simulink model "Q3 – Ramp Signal Folding"  (R2024b)
settings: Solver=FixedStepAuto  StartTime=-5  StopTime=5  FixedStep=0.001  RelTol=1e-3
libraries: simulink x1
settings Model: Creator=sobha  LastModifiedBy=sobha

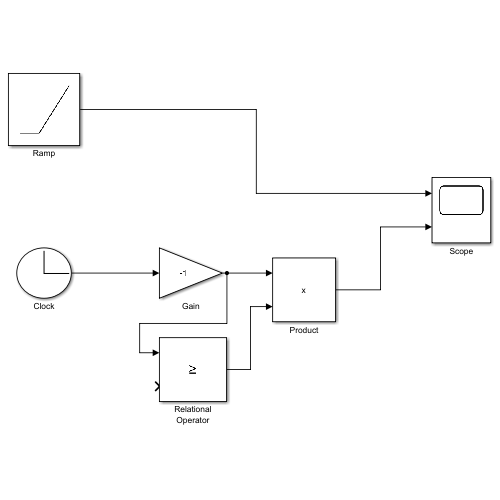
[thumbnail: Simulink's stored preview of the top-level diagram]
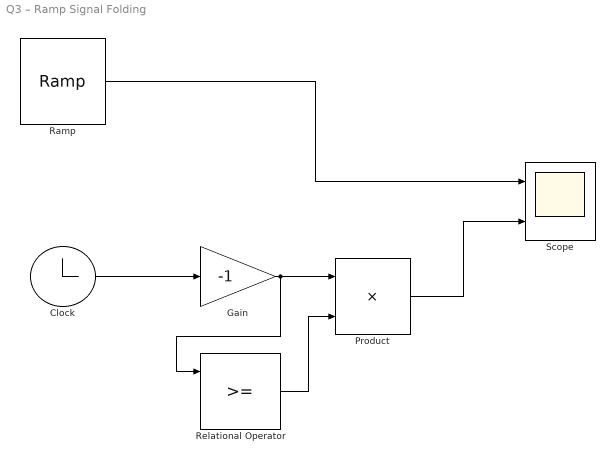
== system Q3 – Ramp Signal Folding ==
  Clock : Clock
  Gain : Gain  Gain=-1
  Product : Product
  Ramp : simulink/Sources/Ramp  slope=1  start=0  InitialOutput=0
  Relational Operator : RelationalOperator  OutDataTypeStr=boolean  RndMeth=Simplest  InputSameDT=off
  Scope : Scope  NumInputPorts=2
  wires:
  Gain/1 -> Relational Operator/1, Product/1
  Clock/1 -> Gain/1
  Ramp/1 -> Scope/1
  Product/1 -> Scope/2
  Relational Operator/1 -> Product/2
